simulink model "q3s"  (R2022a)
settings: Solver=VariableStepAuto  StartTime=0.0  StopTime=2000  RelTol=1e-3
settings Model: Creator=giova  LastModifiedBy=giova

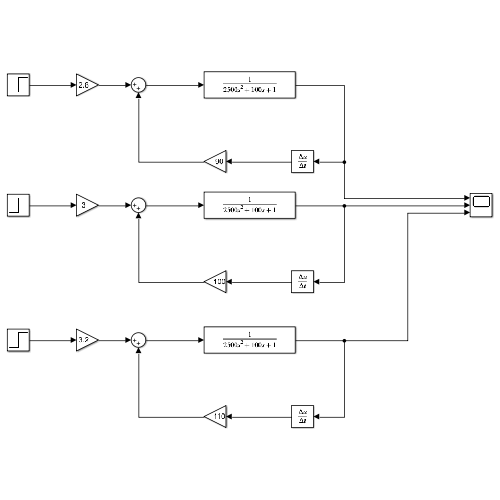
[thumbnail: Simulink's stored preview of the top-level diagram]
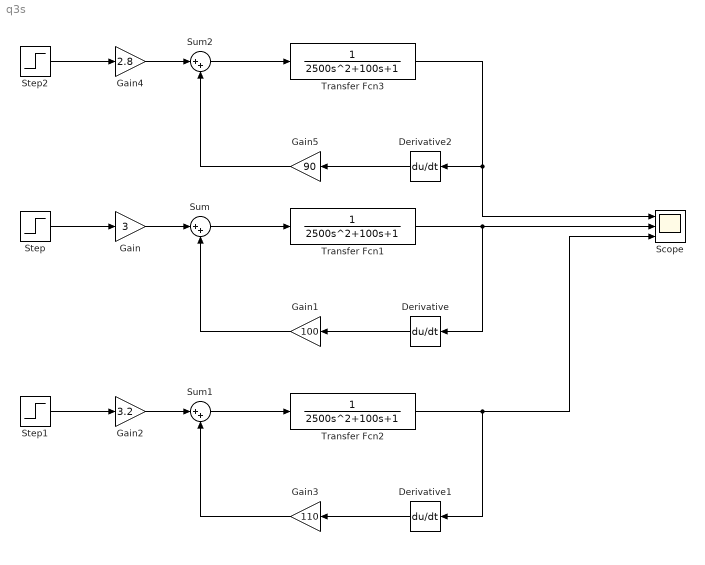
== system q3s ==
  Derivative : Derivative
  Derivative1 : Derivative
  Derivative2 : Derivative
  Gain : Gain  Gain=3
  Gain1 : Gain  Gain=100
  Gain2 : Gain  Gain=3.2
  Gain3 : Gain  Gain=110
  Gain4 : Gain  Gain=2.8
  Gain5 : Gain  Gain=90
  Scope : Scope  NumInputPorts=3
  Step : Step  SampleTime=0
  Step1 : Step  SampleTime=0
  Step2 : Step  SampleTime=0
  Sum : Sum  Inputs=|++
  Sum1 : Sum  Inputs=|++
  Sum2 : Sum  Inputs=|++
  Transfer Fcn1 : TransferFcn  Denominator=[2500 100 1]
  Transfer Fcn2 : TransferFcn  Denominator=[2500 100 1]
  Transfer Fcn3 : TransferFcn  Denominator=[2500 100 1]
  wires:
  Transfer Fcn1/1 -> Scope/2, Derivative/1
  Derivative/1 -> Gain1/1
  Step/1 -> Gain/1
  Sum/1 -> Transfer Fcn1/1
  Gain/1 -> Sum/1
  Gain1/1 -> Sum/2
  Step1/1 -> Gain2/1
  Transfer Fcn2/1 -> Scope/3, Derivative1/1
  Derivative1/1 -> Gain3/1
  Sum1/1 -> Transfer Fcn2/1
  Gain3/1 -> Sum1/2
  Gain2/1 -> Sum1/1
  Step2/1 -> Gain4/1
  Transfer Fcn3/1 -> Scope/1, Derivative2/1
  Derivative2/1 -> Gain5/1
  Sum2/1 -> Transfer Fcn3/1
  Gain5/1 -> Sum2/2
  Gain4/1 -> Sum2/1
